simulink model "block_diagram_ode3"  (R2025b)
settings: Solver=ode8  StartTime=0.0  StopTime=10.0  FixedStep=0.01  RelTol=1e-3
settings Model: Creator=MehrSystem  LastModifiedBy=MehrSystem

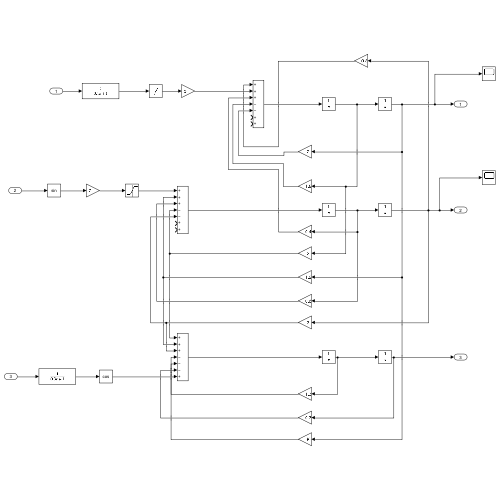
[thumbnail: Simulink's stored preview of the top-level diagram]
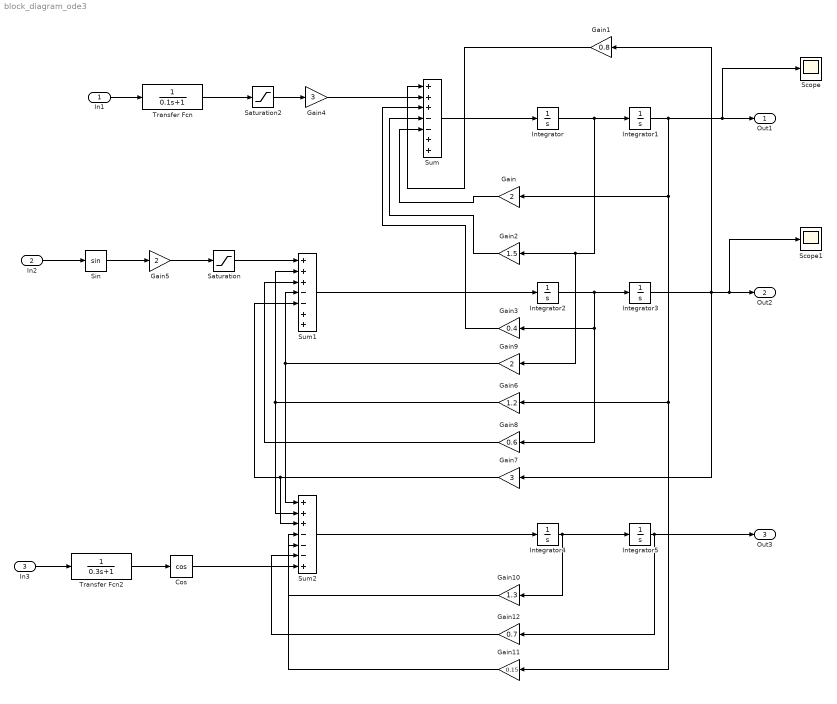
== system block_diagram_ode3 ==
  In1 : Inport
  In2 : Inport  Port=2
  In3 : Inport  Port=3
  Cos : Trigonometry  Operator=cos
  Gain : Gain  Gain=2
  Gain1 : Gain  Gain=0.8
  Gain10 : Gain  Gain=1.3
  Gain11 : Gain  Gain=0.15
  Gain12 : Gain  Gain=0.7
  Gain2 : Gain  Gain=1.5
  Gain3 : Gain  Gain=0.4
  Gain4 : Gain  Gain=3
  Gain5 : Gain  Gain=2
  Gain6 : Gain  Gain=1.2
  Gain7 : Gain  Gain=3
  Gain8 : Gain  Gain=0.6
  Gain9 : Gain  Gain=2
  Integrator{,1..5} (6 alike) : Integrator
  Saturation : Saturate  UpperLimit=0.8  LowerLimit=-1.5
  Saturation2 : Saturate  UpperLimit=2.5  LowerLimit=-0.7
  Scope : Scope
  Scope1 : Scope
  Sin : Trigonometry
  Sum : Sum  Inputs=+++--++
  Sum1 : Sum  Inputs=+++--++
  Sum2 : Sum  Inputs=+++---+
  Transfer Fcn : TransferFcn  Denominator=[0.1 1]
  Transfer Fcn2 : TransferFcn  Denominator=[0.3 1]
  Out1 : Outport
  Out2 : Outport  Port=2
  Out3 : Outport  Port=3
  wires:
  Integrator/1 -> Gain2/1, Gain9/1, Integrator1/1
  Integrator1/1 -> Scope/1, Out1/1, Gain/1, Gain11/1, Gain6/1
  Integrator2/1 -> Gain3/1, Gain8/1, Integrator3/1
  Sum/1 -> Integrator/1
  Gain/1 -> Sum/5
  Integrator3/1 -> Gain1/1, Scope1/1, Out2/1, Gain7/1
  Gain1/1 -> Sum/1
  Gain2/1 -> Sum/4
  Gain3/1 -> Sum/3
  In1/1 -> Transfer Fcn/1
  Gain4/1 -> Sum/2
  Sum1/1 -> Integrator2/1
  In2/1 -> Sin/1
  Gain5/1 -> Saturation/1
  Gain6/1 -> Sum2/2, Sum1/2
  Gain7/1 -> Sum2/3, Sum1/5
  Gain8/1 -> Sum1/3
  Gain9/1 -> Sum2/1, Sum1/4
  Transfer Fcn/1 -> Saturation2/1
  Sin/1 -> Gain5/1
  Integrator4/1 -> Gain10/1, Integrator5/1
  Integrator5/1 -> Gain12/1, Out3/1
  Sum2/1 -> Integrator4/1
  Gain11/1 -> Sum2/4
  Gain10/1 -> Sum2/5
  Gain12/1 -> Sum2/6
  In3/1 -> Transfer Fcn2/1
  Transfer Fcn2/1 -> Cos/1
  Saturation/1 -> Sum1/1
  Cos/1 -> Sum2/7
  Saturation2/1 -> Gain4/1
